simulink model "IEEE39_ClosedLoop"  (R2025a)
settings: Solver=FixedStepDiscrete  StartTime=0.0  StopTime=stopTime  FixedStep=dt  RelTol=1e-3
values from neighbouring files (symbols this model uses):
  dt = double(entry.step_s)    [run_fmu_cosim_sweep.m]    (also in run_ieee39_closed_loop.m; run_ieee39_native_closed_loop.m)
  loadStepTime = double(entry.load_step_s)    [run_ieee39_closed_loop.m]    (also in run_ieee39_native_closed_loop.m)
  stopTime = double(entry.stop_time_s)    [run_fmu_cosim_sweep.m]    (also in run_ieee39_closed_loop.m; run_ieee39_native_closed_loop.m; run_native_replay.m = simulateToTime)
settings Model: Creator=matthiasmees  LastModifiedBy=matthiasmees
settings DataIOCC: SaveOutput=off  SignalLogging=off  SaveTime=off

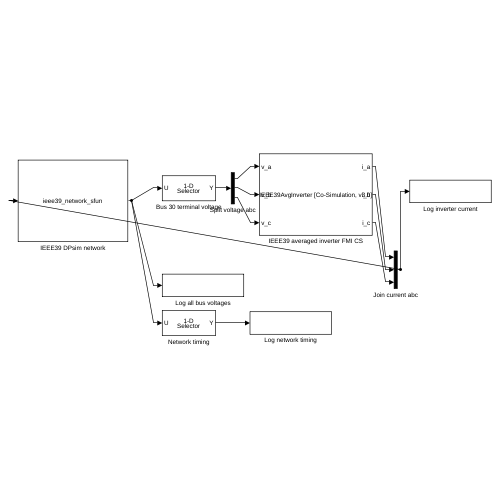
[thumbnail: Simulink's stored preview of the top-level diagram]
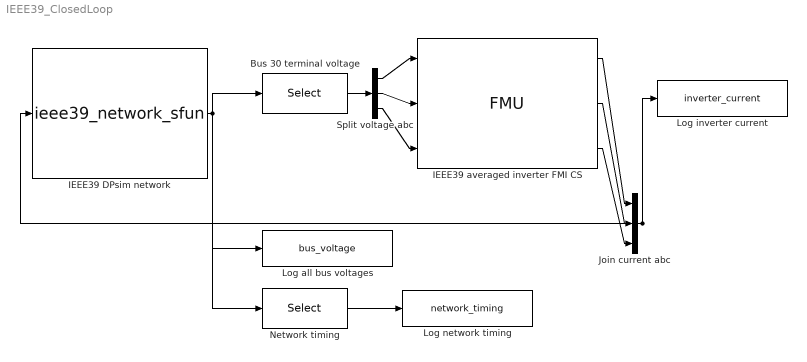
== system IEEE39_ClosedLoop ==
  Bus 30 terminal voltage : Selector  InputPortWidth=119  IndexOptions=Index vector (dialog)  Indices=88:90  OutputSizes=1
  IEEE39 DPsim network : S-Function  FunctionName=ieee39_network_sfun  Parameters=dt,stopTime,loadStepTime  SFunctionDeploymentMode=off  EnableBusSupport=off
  IEEE39 averaged inverter FMI CS : FMU  FMUName=IEEE39AvgInverter.fmu  FMUInputMapping=Flat  FMUOutputMapping=Flat  FMUMode=CoSimulation
      mask Type: IEEE39AvgInverter [Co-Simulation, v3.0]
      mask Display:
      | disp('IEEE39AvgInverter [Co-Simulation, v3.0]');
      | port_label('output',1,'i_a');
      | port_label('output',2,'i_b');
      | port_label('output',3,'i_c');
      | port_label('input',1,'v_a');
      | port_label('input',2,'v_b');
      | port_label('input',3,'v_c');
  Join current abc : Mux  Inputs=3
  Log all bus voltages : ToWorkspace  VariableName=bus_voltage  SaveFormat=Timeseries  SampleTime=-1
  Log inverter current : ToWorkspace  VariableName=inverter_current  SaveFormat=Timeseries  SampleTime=-1
  Log network timing : ToWorkspace  VariableName=network_timing  SaveFormat=Timeseries  SampleTime=-1
  Network timing : Selector  InputPortWidth=119  IndexOptions=Index vector (dialog)  Indices=118:119  OutputSizes=1
  Split voltage abc : Demux  Outputs=3
  wires:
  IEEE39 DPsim network/1 -> Bus 30 terminal voltage/1, Log all bus voltages/1, Network timing/1
  Bus 30 terminal voltage/1 -> Split voltage abc/1
  Split voltage abc/1 -> IEEE39 averaged inverter FMI CS/1
  IEEE39 averaged inverter FMI CS/1 -> Join current abc/1
  Split voltage abc/2 -> IEEE39 averaged inverter FMI CS/2
  IEEE39 averaged inverter FMI CS/2 -> Join current abc/2
  Split voltage abc/3 -> IEEE39 averaged inverter FMI CS/3
  IEEE39 averaged inverter FMI CS/3 -> Join current abc/3
  Join current abc/1 -> IEEE39 DPsim network/1, Log inverter current/1
  Network timing/1 -> Log network timing/1
